simulink model "primero"  (R2023b)
settings: Solver=VariableStepAuto  StartTime=0.0  StopTime=20  RelTol=1e-3
values from neighbouring files (symbols this model uses):
  F = false    [Constantes.m]
  T = true    [Constantes.m]
settings Model: Creator=bruno  LastModifiedBy=bruno

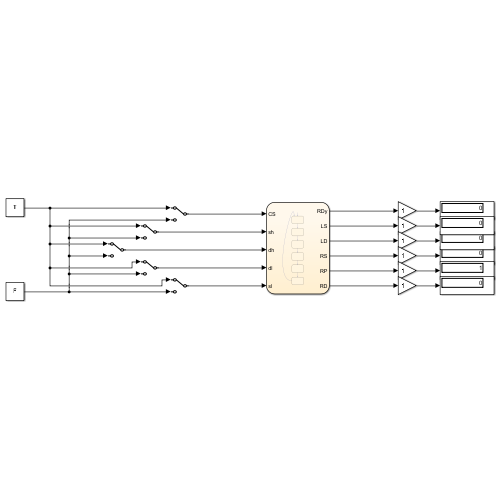
[thumbnail: Simulink's stored preview of the top-level diagram]
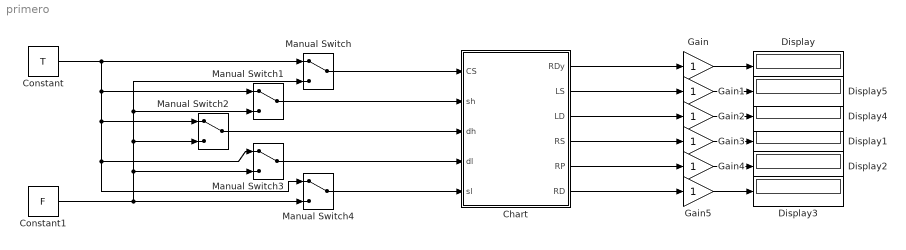
== system primero ==
  Chart : Stateflow chart  TreatAsAtomicUnit=on
  Constant : Constant  Value=T
  Constant1 : Constant  Value=F
  Display{,1..5} (6 alike) : Display
  Gain{,1..5} (6 alike) : Gain
  Manual Switch{,1..4} (5 alike) : ManualSwitch
  wires:
  Chart/1(RDy) -> Gain/1
  Chart/2(LS) -> Gain1/1
  Chart/3(LD) -> Gain2/1
  Chart/4(RS) -> Gain3/1
  Chart/5(RP) -> Gain4/1
  Chart/6(RD) -> Gain5/1
  Manual Switch/1 -> Chart/1(CS)
  Manual Switch1/1 -> Chart/2(sh)
  Manual Switch2/1 -> Chart/3(dh)
  Manual Switch3/1 -> Chart/4(dl)
  Manual Switch4/1 -> Chart/5(sl)
  Constant1/1 -> Manual Switch/2, Manual Switch1/2, Manual Switch2/2, Manual Switch3/2, Manual Switch4/2
  Constant/1 -> Manual Switch/1, Manual Switch4/1, Manual Switch3/1, Manual Switch2/1, Manual Switch1/1
  Gain/1 -> Display/1
  Gain1/1 -> Display5/1
  Gain2/1 -> Display4/1
  Gain3/1 -> Display1/1
  Gain4/1 -> Display2/1
  Gain5/1 -> Display3/1

== stateflow chart primero/Chart ==
  state a
    during:RDy = sh && dh
  state b
    during:LS=true
    RDy=false
  state c
    during:RS=true
    LS=false
  state d
    during:LD=true
    RS=false
  state e
    during:RP=true
    LD=false
  state f
    during:RD=true
    RP=false
  f -> a : [dh]
  (default) -> a
  a -> b : [CS && sh && dh]
  b -> c : [sl]
  c -> d : [sh]
  d -> e : [dl]
  e -> f : [after(5,sec)]
  data: CS input; sh input; dh input; dl input; sl input; RDy output; LS output; LD output; RS output; RP output; RD output
